simulink library "Contact_Forces_Lib"  (R2025a)
settings: Solver=ode45  StartTime=0.0  StopTime=10.0  RelTol=1e-3  EnableMultiTasking=on
undefined symbols (not defined in the file or in its folder): b_contact, custom_param_1, custom_param_2, Extr_Data_Ring, k_contact, l_cone, length_cylinder, length_tube, mu_kinetic, mu_static, pen_exponent, pen_full_damp_F, rad_s_cone, radius_cylinder, radius_tube, v_thr, X, Y, Z
libraries: nesl_utility x197, sm_lib x115, $bdroot x72, simulink x20, fl_lib x4
(part 1 of 12)
Description:
  | Simscape Multibody Contact Forces Library v5.0
  | Copyright 2014-2025 The MathWorks, Inc.
settings Model: Creator=smiller  LastModifiedBy=smiller
settings SolverCC: AlgebraicLoopSolver=TrustRegion
settings DataIOCC: LimitDataPoints=on  SaveFormat=Array  ReturnWorkspaceOutputs=off
settings OptimizationCC: ReuseModelBlockBuffer=off  LifeSpan=inf
settings DebuggingCC: SolverPrmCheckMsg=warning  UnconnectedInputMsg=warning  UnconnectedOutputMsg=warning  UnconnectedLineMsg=warning  AllowSymbolicDim=off  PregeneratedLibrarySubsystemCodeDiagnostic=none  SFUnexpectedBacktrackingDiag=warning  SFNoUnconditionalDefaultTransitionDiag=warning  SFExecutionAtInitializationDiag=none  ArithmeticOperatorsInVariantConditions=warning
settings HardwareCC: ProdBitPerPointer=32.0  ProdBitPerSizeT=32.0  ProdBitPerPtrDiffT=32.0  ProdLargestAtomicFloat=None  ProdIntDivRoundTo=Undefined  ProdEndianess=Unspecified  ProdWordSize=32.0  ProdHWDeviceType=32-bit Generic
settings ModelReferenceCC: EnableRefExpFcnMdlSchedulingChecks=on  PropagateSignalLabelsOutOfModel=off
settings SFSimCC: SimUseLocalCustomCode=off  CustomCodeUndefinedFunction=UseInterfaceOnly
settings RTWCC: RTWUseLocalCustomCode=off  GPUComputeCapability=3.5  DLArmComputeVersion=19.05
settings CodeAppCC: StateflowObjectComments=on
settings GRTTargetCC: TargetLangStandard=C89/C90 (ANSI)
settings ConfigComp: CovMetricSettings=dw  CovSaveCumulativeToWorkspaceVar=on  CovSaveSingleToWorkspaceVar=on  CovExternalEMLEnable=off  CovSFcnEnable=off

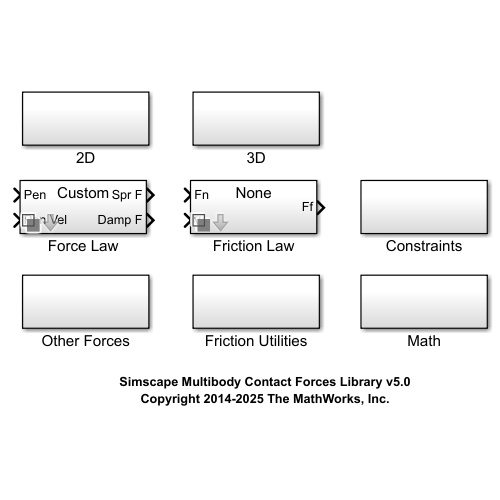
[thumbnail: Simulink's stored preview of the top-level diagram]
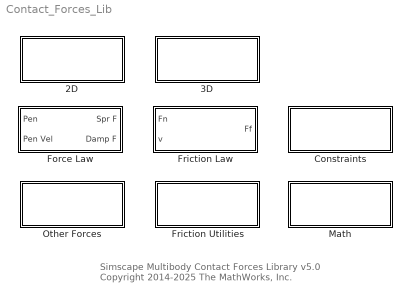
== system Contact_Forces_Lib ==
  note: Simscape Multibody Contact Forces Library v5.0
      | Copyright 2014-2025 The MathWorks, Inc.
  2D : Subsystem
  3D : Subsystem
  Constraints : Subsystem
  Force Law : Subsystem  Variant=on  VariantControlMode=label  LabelModeActiveChoice=Custom
  Friction Law : Subsystem  Variant=on  VariantControlMode=label  LabelModeActiveChoice=None
  Friction Utilities : Subsystem
  Math : Subsystem
  Other Forces : Subsystem

== system Contact_Forces_Lib/2D ==
  Circle to Circle Force : Subsystem  mask(Circle to Circle Force){cirB_rad=0.1, cirF_rad=0.1, active_angle=[-180 180], force_law=Linear, k_contact=1e4, b_contact=1e2, pen_full_damp_F=1e-4, pen_exponent=1, custom_param_1=1, custom_param_2=1, friction_law=None, mu_kinetic=0.5, mu_static=0.7, v_thr=0.001, vis_on=off, vis_opc_en=0, vis_len_cirBz=0.1, vis_len_cirBx=0.005, vis_len_cirFz=0.1, vis_len_cirFx=0.005, vis_clr=[0.9 0.2 0.2], vis_opc=0.7}
      mask prompts: cirB_rad "Base Radius (m)"; cirF_rad "Follower Radius (m)"; active_angle "Active Range (min, max angle (deg))"; force_law "Force Law"; k_contact "Contact Stiffness (N/m)"; b_contact "Contact Damping (N/(m/s))"; pen_full_damp_F "Penetration for full damping (m)"; pen_exponent "Penetration exponent (>=1)"; custom_param_1 "Custom Parameter 1"; custom_param_2 "Custom Parameter 2"; friction_law "Friction Law"; mu_kinetic "Coefficient of Kinetic Friction"; mu_static "Coefficient of Static Friction"; v_thr "Velocity Threshold (m/s)"; vis_on "Visualize Contact Surfaces"; vis_opc_en "Visualize Opacity Enable"; vis_clr "Color of Surface Element (RGB)"; vis_opc "Opacity of Surface Element (0-1)"
      mask help:
      | This subsystem implements a 2D contact force between two circles. It acts to repel frames CirB and CirF.
      |
      | Frames connected to ports:
      | 1. Located at center of circle
      | 2. Circle is in XY plane of frame
      | 3. Active range: counter-clockwise from -x axis of CirB
      |
      | Output signal is a bus with intermediate calculations and total force. Click Help for a diagram describing this force.
      mask init:
      | if strcmp(get_param(gcb,'force_law'),'Linear')
      |     set_param([gcb '/Force Law'],'OverrideUsingVariant','Linear');
      | elseif strcmp(get_param(gcb,'force_law'),'Nonlinear')
      |     set_param([gcb '/Force Law'],'OverrideUsingVariant','Nonlinear');
      | elseif strcmp(get_param(gcb,'force_law'),'Custom')
      |     set_param([gcb '/Force Law'],'OverrideUsingVariant','Custom');
      | end
      | 
      | if strcmp(get_param(gcb,'friction_law'),'None')
      |     set_param([gcb '/Ff/Friction Law'],'OverrideUsingVariant','None');
      | elseif strcmp(get_param(gcb,'friction_law'),'Stick-Slip Continuous')
      |     set_param([gcb '/Ff/Friction Law'],'OverrideUsingVariant','Stick_Slip_C');
      | end
      | 
      | if strcmp(get_param(gcb,'vis_on'),'on')
      |     vis_opc_en = 1;
      | elseif strcmp(get_param(gcb,'vis_on'),'off')
      |     vis_opc_en = 0;
      | end
      mask Help: web(which('Circle_to_Circle_Contact.html'));
      mask TypeOptions force_law: Linear | Nonlinear | Custom
      mask Callback force_law:
      | maskObj = Simulink.Mask.get(gcb);
      | pfd_h = maskObj.getParameter('pen_full_damp_F');
      | pex_h = maskObj.getParameter('pen_exponent');
      | cc1_h = maskObj.getParameter('custom_param_1');
      | cc2_h = maskObj.getParameter('custom_param_2');
      | if strcmp(get_param(gcb,'force_law'),'Linear')
      |     pfd_h.Visible = 'off';
      |     pex_h.Visible = 'off';
      |     cc1_h.Visible = 'off';
      |     cc2_h.Visible = 'off';
      | elseif strcmp(get_param(gcb,'force_law'),'Nonlinear')
      |     pfd_h.Visible = 'on';
      |     pex_h.Visible = 'on';
      |     cc1_h.Visible = 'off';
      |     cc2_h.Visible = 'off';
      | elseif strcmp(get_param(gcb,'force_law'),'Custom')
      |     pfd_h.Visible = 'off';
      |     pex_h.Visible = 'off';
      |     cc1_h.Visible = 'on';
      |     cc2_h.Visible = 'on';
      | end
      | 
      | clear maskObj pfd_h pex_h cc1_h cc2_h
      mask TypeOptions friction_law: None | Stick-Slip Continuous
      mask Callback friction_law:
      | maskObj = Simulink.Mask.get(gcb);
      | muk_h = maskObj.getParameter('mu_kinetic');
      | mus_h = maskObj.getParameter('mu_static');
      | vth_h = maskObj.getParameter('v_thr');
      | if strcmp(get_param(gcb,'friction_law'),'None')
      |     muk_h.Visible = 'off';
      |     mus_h.Visible = 'off';
      |     vth_h.Visible = 'off';
      | elseif strcmp(get_param(gcb,'friction_law'),'Stick-Slip Continuous')
      |     muk_h.Visible = 'on';
      |     mus_h.Visible = 'on';
      |     vth_h.Visible = 'on';
      | end
      | clear maskObj muk_h mus_h vth_h
      mask Callback vis_on:
      | maskObj = Simulink.Mask.get(gcb);
      | 
      | vis_len_prompt_h = maskObj.getDialogControl('vis_len_prompt');
      | vis_len_promptZaxis_h = maskObj.getDialogControl('vis_len_promptZaxis');
      | vis_len_promptXaxis_h = maskObj.getDialogControl('vis_len_promptXaxis');
      | vis_len_promptBase_h = maskObj.getDialogControl('vis_len_promptBase');
      | vis_len_promptFollower_h = maskObj.getDialogControl('vis_len_promptFollower');
      | vis_len_cirBz_h = maskObj.getParameter('vis_len_cirBz');
      | vis_len_cirBx_h = maskObj.getParameter('vis_len_cirBx');
      | vis_len_cirFz_h = maskObj.getParameter('vis_len_cirFz');
      | vis_len_cirFx_h = maskObj.getParameter('vis_len_cirFx');
      | vis_clr_h = maskObj.getParameter('vis_clr');
      | vis_opc_h = maskObj.getParameter('vis_opc');
      | 
      | temp_visCBstate = get_param(gcb,'vis_on');
      | vis_len_prompt_h.Visible = temp_visCBstate;
      | vis_len_promptZaxis_h.Visible = temp_visCBstate;
      | vis_len_promptXaxis_h.Visible = temp_visCBstate;
      | vis_len_promptBase_h.Visible = temp_visCBstate;
      | vis_len_promptFollower_h.Visible = temp_visCBstate;
      | vis_len_cirBz_h.Visible = temp_visCBstate;
      | vis_len_cirBx_h.Visible = temp_visCBstate;
      | vis_len_cirFz_h.Visible = temp_visCBstate;
      | vis_len_cirFx_h.Visible = temp_visCBstate;
      | vis_clr_h.Visible = temp_visCBstate;
      | vis_opc_h.Visible = temp_visCBstate;
      | 
      | clear maskObj vis_clr_h vis_opc_h
      | clear vis_len_prompt_h temp_visCBstate
      | clear vis_len_promptZaxis_h vis_len_promptXaxis_h
      | clear vis_len_promptBase_h vis_len_promptFollower_h
      | clear vis_len_cirBz_h vis_len_cirBx_h
      | clear vis_len_cirFz_h vis_len_cirFx_h
      mask DialogControl Dim_Cont Prompt: Dimensions
      mask DialogControl Con_cont Prompt: Contact
      mask DialogControl Fri_Cont Prompt: Friction
      mask DialogControl Container11 Prompt: Visual
      mask DialogControl vis_len_prompt Prompt: Length of Surface
      mask DialogControl vis_len_promptZaxis Prompt: Z-Axis (m)
      mask DialogControl vis_len_promptXaxis Prompt: X-Axis (m)
      mask DialogControl vis_len_promptBase Prompt: Base
      mask DialogControl vis_len_promptFollower Prompt: Follower
      mask Display: image('Circle_to_Circle_Contact_IMAGE.jpg');
  Circle to Circle Force Enabled : Subsystem  mask(Circle to Circle Force Enabled){cirB_rad=0.1, cirF_rad=0.1, active_angle=[-180 180], force_law=Linear, k_contact=1e4, b_contact=1e2, pen_full_damp_F=1e-4, pen_exponent=1, custom_param_1=1, custom_param_2=1, friction_law=None, mu_kinetic=0.5, mu_static=0.7, v_thr=0.001, vis_on=off, vis_opc_en=0, vis_len_cirBz=0.1, vis_len_cirBx=0.005, vis_len_cirFz=0.1, vis_len_cirFx=0.005, vis_clr=[0.9 0.2 0.2], vis_opc=0.7}
      mask prompts: cirB_rad "Base Radius (m)"; cirF_rad "Follower Radius (m)"; active_angle "Active Range (min, max angle (deg))"; force_law "Force Law"; k_contact "Contact Stiffness (N/m)"; b_contact "Contact Damping (N/(m/s))"; pen_full_damp_F "Penetration for full damping (m)"; pen_exponent "Penetration exponent (>=1)"; custom_param_1 "Custom Parameter 1"; custom_param_2 "Custom Parameter 2"; friction_law "Friction Law"; mu_kinetic "Coefficient of Kinetic Friction"; mu_static "Coefficient of Static Friction"; v_thr "Velocity Threshold (m/s)"; vis_on "Visualize Contact Surfaces"; vis_opc_en "Visualize Opacity Enable"; vis_clr "Color of Surface Element (RGB)"; vis_opc "Opacity of Surface Element (0-1)"
      mask help:
      | This subsystem implements a 2D contact force between two circles. It acts to repel frames CirB and CirF.
      |
      | Frames connected to ports:
      | 1. Located at center of circle
      | 2. Circle is in XY plane of frame
      | 3. Active range: counter-clockwise from -x axis of CirB
      |
      | Input signal is a bus with signals that control aspects of the force, including enable/disable. Output signal is a bus with intermediate calculations and total force. Click Help for a diagram describing this force.
      mask init: same as Contact_Forces_Lib/2D/Circle to Circle Force
      mask Help: web(which('Circle_to_Circle_Contact.html'));
      mask TypeOptions force_law: Linear | Nonlinear | Custom
      mask Callback force_law:
      | maskObj = Simulink.Mask.get(gcb);
      | pfd_h = maskObj.getParameter('pen_full_damp_F');
      | pex_h = maskObj.getParameter('pen_exponent');
      | cc1_h = maskObj.getParameter('custom_param_1');
      | cc2_h = maskObj.getParameter('custom_param_2');
      | if strcmp(get_param(gcb,'force_law'),'Linear')
      |     pfd_h.Visible = 'off';
      |     pex_h.Visible = 'off';
      |     cc1_h.Visible = 'off';
      |     cc2_h.Visible = 'off';
      | elseif strcmp(get_param(gcb,'force_law'),'Nonlinear')
      |     pfd_h.Visible = 'on';
      |     pex_h.Visible = 'on';
      |     cc1_h.Visible = 'off';
      |     cc2_h.Visible = 'off';
      | elseif strcmp(get_param(gcb,'force_law'),'Custom')
      |     pfd_h.Visible = 'off';
      |     pex_h.Visible = 'off';
      |     cc1_h.Visible = 'on';
      |     cc2_h.Visible = 'on';
      | end
      | 
      | clear maskObj pfd_h pex_h cc1_h cc2_h
      mask TypeOptions friction_law: None | Stick-Slip Continuous
      mask Callback friction_law:
      | maskObj = Simulink.Mask.get(gcb);
      | muk_h = maskObj.getParameter('mu_kinetic');
      | mus_h = maskObj.getParameter('mu_static');
      | vth_h = maskObj.getParameter('v_thr');
      | if strcmp(get_param(gcb,'friction_law'),'None')
      |     muk_h.Visible = 'off';
      |     mus_h.Visible = 'off';
      |     vth_h.Visible = 'off';
      | elseif strcmp(get_param(gcb,'friction_law'),'Stick-Slip Continuous')
      |     muk_h.Visible = 'on';
      |     mus_h.Visible = 'on';
      |     vth_h.Visible = 'on';
      | end
      | clear maskObj muk_h mus_h vth_h
      mask Callback vis_on:
      | maskObj = Simulink.Mask.get(gcb);
      | 
      | vis_len_prompt_h = maskObj.getDialogControl('vis_len_prompt');
      | vis_len_promptZaxis_h = maskObj.getDialogControl('vis_len_promptZaxis');
      | vis_len_promptXaxis_h = maskObj.getDialogControl('vis_len_promptXaxis');
      | vis_len_promptBase_h = maskObj.getDialogControl('vis_len_promptBase');
      | vis_len_promptFollower_h = maskObj.getDialogControl('vis_len_promptFollower');
      | vis_len_cirBz_h = maskObj.getParameter('vis_len_cirBz');
      | vis_len_cirBx_h = maskObj.getParameter('vis_len_cirBx');
      | vis_len_cirFz_h = maskObj.getParameter('vis_len_cirFz');
      | vis_len_cirFx_h = maskObj.getParameter('vis_len_cirFx');
      | vis_clr_h = maskObj.getParameter('vis_clr');
      | vis_opc_h = maskObj.getParameter('vis_opc');
      | 
      | temp_visCBstate = get_param(gcb,'vis_on');
      | vis_len_prompt_h.Visible = temp_visCBstate;
      | vis_len_promptZaxis_h.Visible = temp_visCBstate;
      | vis_len_promptXaxis_h.Visible = temp_visCBstate;
      | vis_len_promptBase_h.Visible = temp_visCBstate;
      | vis_len_promptFollower_h.Visible = temp_visCBstate;
      | vis_len_cirBz_h.Visible = temp_visCBstate;
      | vis_len_cirBx_h.Visible = temp_visCBstate;
      | vis_len_cirFz_h.Visible = temp_visCBstate;
      | vis_len_cirFx_h.Visible = temp_visCBstate;
      | vis_clr_h.Visible = temp_visCBstate;
      | vis_opc_h.Visible = temp_visCBstate;
      | 
      | clear maskObj vis_clr_h vis_opc_h
      | clear vis_len_prompt_h temp_visCBstate
      | clear vis_len_promptZaxis_h vis_len_promptXaxis_h
      | clear vis_len_promptBase_h vis_len_promptFollower_h
      | clear vis_len_cirBz_h vis_len_cirBx_h
      | clear vis_len_cirFz_h vis_len_cirFx_h
      mask DialogControl Dim_Cont Prompt: Dimensions
      mask DialogControl Con_cont Prompt: Contact
      mask DialogControl Fri_Cont Prompt: Friction
      mask DialogControl Container11 Prompt: Visual
      mask DialogControl vis_len_prompt Prompt: Length of Surface
      mask DialogControl vis_len_promptZaxis Prompt: Z-Axis (m)
      mask DialogControl vis_len_promptXaxis Prompt: X-Axis (m)
      mask DialogControl vis_len_promptBase Prompt: Base
      mask DialogControl vis_len_promptFollower Prompt: Follower
      mask Display: image('Circle_to_Circle_Contact_Enabled_IMAGE.jpg');
  Circle to Finite Line Force : Subsystem  mask(Circle on Finite Line Force){circle_rad=0.2, line_depth=0.05/2, line_length=5, force_law=Linear, k_contact=1e5, b_contact=1e2, pen_full_damp_F=1e-4, pen_exponent=1, custom_param_1=1, custom_param_2=1, friction_law=None, mu_kinetic=0.5, mu_static=0.7, v_thr=0.001, vis_on=off, vis_opc_en=0, vis_len_linBz=0.1, vis_len_linBx=0.005, vis_len_cirFz=0.1, vis_len_cirFx=0.005, vis_clr=[0.9 0.2 0.2], vis_opc=0.7}
      mask prompts: circle_rad "Circle Radius (m)"; line_depth "Line Depth to Reference Frame (m)"; line_length "Line Length (m)"; force_law "Force Law"; k_contact "Contact Stiffness (N/m)"; b_contact "Contact Damping (N/(m/s))"; pen_full_damp_F "Penetration for full damping (m)"; pen_exponent "Penetration exponent (>=1)"; custom_param_1 "Custom Parameter 1"; custom_param_2 "Custom Parameter 2"; friction_law "Friction Law"; mu_kinetic "Coefficient of Kinetic Friction"; mu_static "Coefficient of Static Friction"; v_thr "Velocity Threshold (m/s)"; vis_on "Visualize Contact Surface"; vis_opc_en "Visualize Opacity Enable"; vis_clr "Color of Surface Element (RGB)"; vis_opc "Opacity of Surface Element (0-1)"
      mask help:
      | This subsystem implements a 2D contact force between a circle and a finite line.  The force is active above and below the line.
      |
      | Frame connected to LinB port:
      | 1. Located at midpoint of line.
      | 2. X-axis is normal to the finite line.
      | 3. Y-axis is along the finite line.
      |
      | Frame connected to the CirF port:
      | 1. Z-axis aligned with frame attached to LinB port.
      |
      | Output signal is a bus with intermediate calculations and total force. Click Help for a diagram describing this force.
      mask init:
      | if strcmp(get_param(gcb,'force_law'),'Linear')
      |     set_param([gcb '/Forces/Force Law'],'OverrideUsingVariant','Linear');
      | elseif strcmp(get_param(gcb,'force_law'),'Nonlinear')
      |     set_param([gcb '/Forces/Force Law'],'OverrideUsingVariant','Nonlinear');
      | elseif strcmp(get_param(gcb,'force_law'),'Custom')
      |     set_param([gcb '/Forces/Force Law'],'OverrideUsingVariant','Custom');
      | end
      | 
      | if strcmp(get_param(gcb,'friction_law'),'None')
      |     set_param([gcb '/Forces/Resolve Forces/Friction/Friction Law'],'OverrideUsingVariant','None');
      | elseif strcmp(get_param(gcb,'friction_law'),'Stick-Slip Continuous')
      |     set_param([gcb '/Forces/Resolve Forces/Friction/Friction Law'],'OverrideUsingVariant','Stick_Slip_C');
      | end
      | 
      | if strcmp(get_param(gcb,'vis_on'),'on')
      |     vis_opc_en = 1;
      | elseif strcmp(get_param(gcb,'vis_on'),'off')
      |     vis_opc_en = 0;
      | end
      mask Help: web(which('Circle_to_Finite_Line_Contact.html'));
      mask TypeOptions force_law: Linear | Nonlinear | Custom
      mask Callback force_law:
      | %maskStr = get_param(gcb,'MaskValues');
      | maskObj = Simulink.Mask.get(gcb);
      | pfd_h = maskObj.getParameter('pen_full_damp_F');
      | pex_h = maskObj.getParameter('pen_exponent');
      | cc1_h = maskObj.getParameter('custom_param_1');
      | cc2_h = maskObj.getParameter('custom_param_2');
      | if strcmp(get_param(gcb,'force_law'),'Linear')
      |     pfd_h.Visible = 'off';
      |     pex_h.Visible = 'off';
      |     cc1_h.Visible = 'off';
      |     cc2_h.Visible = 'off';
      | %    set_param(gcb,'MaskVisibilities',{'on' 'on' 'on' 'on' 'on' 'off' 'off' 'off' 'off'});
      | %    set_param(gcb,'MaskVisibilities',{'on' 'on' 'on' 'on' 'on' 'off' 'off' 'off' 'off'});
      | elseif strcmp(get_param(gcb,'force_law'),'Nonlinear')
      |     pfd_h.Visible = 'on';
      |     pex_h.Visible = 'on';
      |     cc1_h.Visible = 'off';
      |     cc2_h.Visible = 'off';
      |     %set_param(gcb,'MaskVisibilities',{'on' 'on' 'on' 'on' 'on' 'on' 'on' 'off' 'off'});
      | elseif strcmp(get_param(gcb,'force_law'),'Custom')
      |     pfd_h.Visible = 'off';
      |     pex_h.Visible = 'off';
      |     cc1_h.Visible = 'on';
      |     cc2_h.Visible = 'on';
      |     %set_param(gcb,'MaskVisibilities',{'on' 'on' 'on' 'on' 'on' 'off' 'off' 'on' 'on'});
      | end
      | %clear maskObj
      | 
      | %maskObj = Simulink.Mask.get(gcb);
      | %if strcmp(get_param(gcb,'x'),'on')
      | %else
      | %    yh.Visible = 'off';
      | %end
      mask TypeOptions friction_law: None | Stick-Slip Continuous
      mask Callback friction_law:
      | maskObj = Simulink.Mask.get(gcb);
      | muk_h = maskObj.getParameter('mu_kinetic');
      | mus_h = maskObj.getParameter('mu_static');
      | vth_h = maskObj.getParameter('v_thr');
      | if strcmp(get_param(gcb,'friction_law'),'None')
      |     muk_h.Visible = 'off';
      |     mus_h.Visible = 'off';
      |     vth_h.Visible = 'off';
      | elseif strcmp(get_param(gcb,'friction_law'),'Stick-Slip Continuous')
      |     muk_h.Visible = 'on';
      |     mus_h.Visible = 'on';
      |     vth_h.Visible = 'on';
      | end
      | clear maskObj
      mask Callback vis_on:
      | maskObj = Simulink.Mask.get(gcb);
      | vis_len_prompt_h = maskObj.getDialogControl('vis_len_prompt');
      | vis_len_promptZaxis_h = maskObj.getDialogControl('vis_len_promptZaxis');
      | vis_len_promptXaxis_h = maskObj.getDialogControl('vis_len_promptXaxis');
      | vis_len_promptBase_h = maskObj.getDialogControl('vis_len_promptBase');
      | vis_len_promptFollower_h = maskObj.getDialogControl('vis_len_promptFollower');
      | vis_len_linBz_h = maskObj.getParameter('vis_len_linBz');
      | vis_len_linBx_h = maskObj.getParameter('vis_len_linBx');
      | vis_len_cirFz_h = maskObj.getParameter('vis_len_cirFz');
      | vis_len_cirFx_h = maskObj.getParameter('vis_len_cirFx');
      | vis_clr_h = maskObj.getParameter('vis_clr');
      | vis_opc_h = maskObj.getParameter('vis_opc');
      | 
      | temp_visCBstate = get_param(gcb,'vis_on');
      | vis_len_prompt_h.Visible = temp_visCBstate;
      | vis_len_promptZaxis_h.Visible = temp_visCBstate;
      | vis_len_promptXaxis_h.Visible = temp_visCBstate;
      | vis_len_promptBase_h.Visible = temp_visCBstate;
      | vis_len_promptFollower_h.Visible = temp_visCBstate;
      | vis_len_linBz_h.Visible = temp_visCBstate;
      | vis_len_linBx_h.Visible = temp_visCBstate;
      | vis_len_cirFz_h.Visible = temp_visCBstate;
      | vis_len_cirFx_h.Visible = temp_visCBstate;
      | vis_clr_h.Visible = temp_visCBstate;
      | vis_opc_h.Visible = temp_visCBstate;
      | 
      | clear maskObj vis_len_h vis_clr_h vis_opc_h
      | clear temp_visCBstate
      | clear vis_len_prompt_h vis_len_promptZaxis_h vis_len_promptXaxis_h
      | clear vis_len_promptBase_h vis_len_promptFollower_h
      | clear vis_len_linBz_h vis_len_linBx_h
      | clear vis_len_cirFz_h vis_len_cirFx_h
      mask DialogControl Dim_Cont Prompt: Dimensions
      mask DialogControl Con_Cont Prompt: Contact
      mask DialogControl Fri_Cont Prompt: Friction
      mask DialogControl Container9 Prompt: Visual
      mask DialogControl vis_len_prompt Prompt: Length of Surface
      mask DialogControl vis_len_promptZaxis Prompt: Z-Axis (m)
      mask DialogControl vis_len_promptXaxis Prompt: X-Axis (m)
      mask DialogControl vis_len_promptBase Prompt: Base (Line)
      mask DialogControl vis_len_promptFollower Prompt: Follower (Cir)
      mask Display: image('Circle_to_Finite_Line_Contact_IMAGE.jpg');
  Circle to Finite Line Force Enabled : Subsystem  mask(Circle on Finite Line Force Enabled){circle_rad=0.2, line_depth=0.05/2, line_length=5, force_law=Linear, k_contact=1e5, b_contact=1e2, pen_full_damp_F=1e-4, pen_exponent=1, custom_param_1=1, custom_param_2=1, friction_law=None, mu_kinetic=0.5, mu_static=0.7, v_thr=0.001, vis_on=off, vis_opc_en=0, vis_len_linBz=0.1, vis_len_linBx=0.005, vis_len_cirFz=0.1, vis_len_cirFx=0.005, vis_clr=[0.9 0.2 0.2], vis_opc=0.7}
      mask prompts: circle_rad "Circle Radius (m)"; line_depth "Line Depth to Reference Frame (m)"; line_length "Line Length (m)"; force_law "Force Law"; k_contact "Contact Stiffness (N/m)"; b_contact "Contact Damping (N/(m/s))"; pen_full_damp_F "Penetration for full damping (m)"; pen_exponent "Penetration exponent (>=1)"; custom_param_1 "Custom Parameter 1"; custom_param_2 "Custom Parameter 2"; friction_law "Friction Law"; mu_kinetic "Coefficient of Kinetic Friction"; mu_static "Coefficient of Static Friction"; v_thr "Velocity Threshold (m/s)"; vis_on "Visualize Contact Surface"; vis_opc_en "Visualize Opacity Enable"; vis_clr "Color of Surface Element (RGB)"; vis_opc "Opacity of Surface Element (0-1)"
      mask help:
      | This subsystem implements a 2D contact force between a circle and a finite line.  The force is active above and below the line.
      |
      | Frame connected to LinB port:
      | 1. Located at midpoint of line.
      | 2. X-axis is normal to the finite line.
      | 3. Y-axis is along the finite line.
      |
      | Frame connected to the CirF port:
      | 1. Z-axis aligned with frame attached to LinB port.
      |
      | Input signal is a bus with signals that control aspects of the force, including enable/disable. Output signal is a bus with intermediate calculations and total force. Click Help for a diagram describing this force.
      mask init: same as Contact_Forces_Lib/2D/Circle to Finite Line Force
      mask Help: web(which('Circle_to_Finite_Line_Contact.html'));
      mask TypeOptions force_law: Linear | Nonlinear | Custom
      mask Callback force_law:
      | %maskStr = get_param(gcb,'MaskValues');
      | maskObj = Simulink.Mask.get(gcb);
      | pfd_h = maskObj.getParameter('pen_full_damp_F');
      | pex_h = maskObj.getParameter('pen_exponent');
      | cc1_h = maskObj.getParameter('custom_param_1');
      | cc2_h = maskObj.getParameter('custom_param_2');
      | if strcmp(get_param(gcb,'force_law'),'Linear')
      |     pfd_h.Visible = 'off';
      |     pex_h.Visible = 'off';
      |     cc1_h.Visible = 'off';
      |     cc2_h.Visible = 'off';
      | %    set_param(gcb,'MaskVisibilities',{'on' 'on' 'on' 'on' 'on' 'off' 'off' 'off' 'off'});
      | %    set_param(gcb,'MaskVisibilities',{'on' 'on' 'on' 'on' 'on' 'off' 'off' 'off' 'off'});
      | elseif strcmp(get_param(gcb,'force_law'),'Nonlinear')
      |     pfd_h.Visible = 'on';
      |     pex_h.Visible = 'on';
      |     cc1_h.Visible = 'off';
      |     cc2_h.Visible = 'off';
      |     %set_param(gcb,'MaskVisibilities',{'on' 'on' 'on' 'on' 'on' 'on' 'on' 'off' 'off'});
      | elseif strcmp(get_param(gcb,'force_law'),'Custom')
      |     pfd_h.Visible = 'off';
      |     pex_h.Visible = 'off';
      |     cc1_h.Visible = 'on';
      |     cc2_h.Visible = 'on';
      |     %set_param(gcb,'MaskVisibilities',{'on' 'on' 'on' 'on' 'on' 'off' 'off' 'on' 'on'});
      | end
      | %clear maskObj
      | 
      | %maskObj = Simulink.Mask.get(gcb);
      | %if strcmp(get_param(gcb,'x'),'on')
      | %else
      | %    yh.Visible = 'off';
      | %end
      mask TypeOptions friction_law: None | Stick-Slip Continuous
      mask Callback friction_law:
      | maskObj = Simulink.Mask.get(gcb);
      | muk_h = maskObj.getParameter('mu_kinetic');
      | mus_h = maskObj.getParameter('mu_static');
      | vth_h = maskObj.getParameter('v_thr');
      | if strcmp(get_param(gcb,'friction_law'),'None')
      |     muk_h.Visible = 'off';
      |     mus_h.Visible = 'off';
      |     vth_h.Visible = 'off';
      | elseif strcmp(get_param(gcb,'friction_law'),'Stick-Slip Continuous')
      |     muk_h.Visible = 'on';
      |     mus_h.Visible = 'on';
      |     vth_h.Visible = 'on';
      | end
      | clear maskObj
      mask Callback vis_on:
      | maskObj = Simulink.Mask.get(gcb);
      | vis_len_prompt_h = maskObj.getDialogControl('vis_len_prompt');
      | vis_len_promptZaxis_h = maskObj.getDialogControl('vis_len_promptZaxis');
      | vis_len_promptXaxis_h = maskObj.getDialogControl('vis_len_promptXaxis');
      | vis_len_promptBase_h = maskObj.getDialogControl('vis_len_promptBase');
      | vis_len_promptFollower_h = maskObj.getDialogControl('vis_len_promptFollower');
      | vis_len_linBz_h = maskObj.getParameter('vis_len_linBz');
      | vis_len_linBx_h = maskObj.getParameter('vis_len_linBx');
      | vis_len_cirFz_h = maskObj.getParameter('vis_len_cirFz');
      | vis_len_cirFx_h = maskObj.getParameter('vis_len_cirFx');
      | vis_clr_h = maskObj.getParameter('vis_clr');
      | vis_opc_h = maskObj.getParameter('vis_opc');
      | 
      | temp_visCBstate = get_param(gcb,'vis_on');
      | vis_len_prompt_h.Visible = temp_visCBstate;
      | vis_len_promptZaxis_h.Visible = temp_visCBstate;
      | vis_len_promptXaxis_h.Visible = temp_visCBstate;
      | vis_len_promptBase_h.Visible = temp_visCBstate;
      | vis_len_promptFollower_h.Visible = temp_visCBstate;
      | vis_len_linBz_h.Visible = temp_visCBstate;
      | vis_len_linBx_h.Visible = temp_visCBstate;
      | vis_len_cirFz_h.Visible = temp_visCBstate;
      | vis_len_cirFx_h.Visible = temp_visCBstate;
      | vis_clr_h.Visible = temp_visCBstate;
      | vis_opc_h.Visible = temp_visCBstate;
      | 
      | clear maskObj vis_len_h vis_clr_h vis_opc_h
      | clear temp_visCBstate
      | clear vis_len_prompt_h vis_len_promptZaxis_h vis_len_promptXaxis_h
      | clear vis_len_promptBase_h vis_len_promptFollower_h
      | clear vis_len_linBz_h vis_len_linBx_h
      | clear vis_len_cirFz_h vis_len_cirFx_h
      mask DialogControl Dim_Cont Prompt: Dimensions
      mask DialogControl Con_Cont Prompt: Contact
      mask DialogControl Fri_Cont Prompt: Friction
      mask DialogControl Container9 Prompt: Visual
      mask DialogControl vis_len_prompt Prompt: Length of Surface
      mask DialogControl vis_len_promptZaxis Prompt: Z-Axis (m)
      mask DialogControl vis_len_promptXaxis Prompt: X-Axis (m)
      mask DialogControl vis_len_promptBase Prompt: Base (Line)
      mask DialogControl vis_len_promptFollower Prompt: Follower (Cir)
      mask Display: image('Circle_to_Finite_Line_Contact_Enabled_IMAGE.jpg');
  Circle to Hole Force : Subsystem  mask(Circle to Hole Force){k_contact=-1e4, b_contact=10, max_frame_sep=0.1079, active_angle=[-180 180], h_deadzone=0.6667}
      mask prompts: k_contact "Attraction Stiffness (N/m)"; b_contact "Attraction Damping (N/(m/s))"; max_frame_sep "Maximum Frame Separation (m)"; active_angle "Active Range (min, max angle relative to frame CirB (deg))"; h_deadzone "Hole Deadzone (% of radius)"
      mask help: This subsystem implements an attraction force between a circle and a hole. This force operates on the XY plane of the CirB frame. A deadzone is applied to the stiffness force at the center of the hole to allow the circle to come to rest.
      mask Display: image('Circle_to_Hole_Attraction_IMAGE.jpg');
  Circle to Ring Force : Subsystem  mask(Circle to Ring Force){radius_circle=0.05, radius_ring=0.07, d_ring=0.02, active_angle=[-120 120], force_law=Linear, k_contact=1e4, b_contact=1e2, pen_full_damp_F=1e-4, pen_exponent=1, custom_param_1=1, custom_param_2=1, friction_law=Stick-Slip Continuous, mu_kinetic=0.1, mu_static=0.2, v_thr=0.001, vis_on=off, vis_opc_en=0, vis_len_rinBz=0.05*1.05, vis_len_rinBx=0.08*0.05, vis_len_cirFz=0.05*1.05, vis_len_cirFx=0.05*0.05, vis_clr=[0.9 0.2 0.2], vis_opc=0.7}
      mask prompts: radius_circle "Circle Radius (CirF) (m)"; radius_ring "Ring Radius (RinB) (m)"; d_ring "Ring Thickness (RinB) (m)"; active_angle "Active Range (min, max angle (deg))"; force_law "Force Law"; k_contact "Contact Stiffness (N/m)"; b_contact "Contact Damping (N/(m/s))"; pen_full_damp_F "Penetration for full damping (m)"; pen_exponent "Penetration exponent (>=1)"; custom_param_1 "Custom Parameter 1"; custom_param_2 "Custom Parameter 2"; friction_law "Friction Law"; mu_kinetic "Coefficient of Kinetic Friction"; mu_static "Coefficient of Static Friction"; v_thr "Velocity Threshold (m/s)"; vis_on "Visualize Contact Surface"; vis_opc_en "Visualize Opacity Enable"; vis_clr "Color of Visual Element (RGB)"; vis_opc "Opacity of Visual Element (0-1)"
      mask help:
      | This subsystem implements a 2D contact force between a circle and a ring.
      | The force is active on the outside and the inside of the ring.
      |
      | Frames connected to ports:
      | 1. Located at center of circle/ring
      | 2. Circle/Ring is in XY plane of frame
      | 3. Active range: relative to +x axis of RinB [-180 180]
      |
      | Output signal is a bus with intermediate calculations and total force. Click Help for a diagram describing this force.
      mask init:
      | if strcmp(get_param(gcb,'force_law'),'Linear')
      |     set_param([gcb '/Forces/Force Law'],'OverrideUsingVariant','Linear');
      | elseif strcmp(get_param(gcb,'force_law'),'Nonlinear')
      |     set_param([gcb '/Forces/Force Law'],'OverrideUsingVariant','Nonlinear');
      | elseif strcmp(get_param(gcb,'force_law'),'Custom')
      |     set_param([gcb '/Forces/Force Law'],'OverrideUsingVariant','Custom');
      | end
      | 
      | if strcmp(get_param(gcb,'friction_law'),'None')
      |     set_param([gcb '/Forces/Ff/Friction Law'],'OverrideUsingVariant','None');
      | elseif strcmp(get_param(gcb,'friction_law'),'Stick-Slip Continuous')
      |     set_param([gcb '/Forces/Ff/Friction Law'],'OverrideUsingVariant','Stick_Slip_C');
      | end
      | 
      | if strcmp(get_param(gcb,'vis_on'),'on')
      |     vis_opc_en = 1;
      | elseif strcmp(get_param(gcb,'vis_on'),'off')
      |     vis_opc_en = 0;
      | end
      mask Help: web(which('Circle_to_Ring_Contact.html'));
      mask TypeOptions force_law: Linear | Nonlinear | Custom
      mask Callback force_law:
      | %maskStr = get_param(gcb,'MaskValues');
      | maskObj = Simulink.Mask.get(gcb);
      | pfd_h = maskObj.getParameter('pen_full_damp_F');
      | pex_h = maskObj.getParameter('pen_exponent');
      | cc1_h = maskObj.getParameter('custom_param_1');
      | cc2_h = maskObj.getParameter('custom_param_2');
      | if strcmp(get_param(gcb,'force_law'),'Linear')
      |     pfd_h.Visible = 'off';
      |     pex_h.Visible = 'off';
      |     cc1_h.Visible = 'off';
      |     cc2_h.Visible = 'off';
      | %    set_param(gcb,'MaskVisibilities',{'on' 'on' 'on' 'on' 'on' 'off' 'off' 'off' 'off'});
      | %    set_param(gcb,'MaskVisibilities',{'on' 'on' 'on' 'on' 'on' 'off' 'off' 'off' 'off'});
      | elseif strcmp(get_param(gcb,'force_law'),'Nonlinear')
      |     pfd_h.Visible = 'on';
      |     pex_h.Visible = 'on';
      |     cc1_h.Visible = 'off';
      |     cc2_h.Visible = 'off';
      |     %set_param(gcb,'MaskVisibilities',{'on' 'on' 'on' 'on' 'on' 'on' 'on' 'off' 'off'});
      | elseif strcmp(get_param(gcb,'force_law'),'Custom')
      |     pfd_h.Visible = 'off';
      |     pex_h.Visible = 'off';
      |     cc1_h.Visible = 'on';
      |     cc2_h.Visible = 'on';
      |     %set_param(gcb,'MaskVisibilities',{'on' 'on' 'on' 'on' 'on' 'off' 'off' 'on' 'on'});
      | end
      | %clear maskObj
      | 
      | %maskObj = Simulink.Mask.get(gcb);
      | %if strcmp(get_param(gcb,'x'),'on')
      | %else
      | %    yh.Visible = 'off';
      | %end
      mask TypeOptions friction_law: None | Stick-Slip Continuous
      mask Callback friction_law:
      | maskObj = Simulink.Mask.get(gcb);
      | muk_h = maskObj.getParameter('mu_kinetic');
      | mus_h = maskObj.getParameter('mu_static');
      | vth_h = maskObj.getParameter('v_thr');
      | if strcmp(get_param(gcb,'friction_law'),'None')
      |     muk_h.Visible = 'off';
      |     mus_h.Visible = 'off';
      |     vth_h.Visible = 'off';
      | elseif strcmp(get_param(gcb,'friction_law'),'Stick-Slip Continuous')
      |     muk_h.Visible = 'on';
      |     mus_h.Visible = 'on';
      |     vth_h.Visible = 'on';
      | end
      | clear maskObj
      mask Callback vis_on:
      | maskObj = Simulink.Mask.get(gcb);
      | 
      | vis_len_prompt_h = maskObj.getDialogControl('vis_len_prompt');
      | vis_len_promptZaxis_h = maskObj.getDialogControl('vis_len_promptZaxis');
      | vis_len_promptXaxis_h = maskObj.getDialogControl('vis_len_promptXaxis');
      | vis_len_promptBase_h = maskObj.getDialogControl('vis_len_promptBase');
      | vis_len_promptFollower_h = maskObj.getDialogControl('vis_len_promptFollower');
      | vis_len_rinBz_h = maskObj.getParameter('vis_len_rinBz');
      | vis_len_rinBx_h = maskObj.getParameter('vis_len_rinBx');
      | vis_len_cirFz_h = maskObj.getParameter('vis_len_cirFz');
      | vis_len_cirFx_h = maskObj.getParameter('vis_len_cirFx');
      | vis_clr_h = maskObj.getParameter('vis_clr');
      | vis_opc_h = maskObj.getParameter('vis_opc');
      | 
      | temp_visCBstate = get_param(gcb,'vis_on');
      | vis_len_prompt_h.Visible = temp_visCBstate;
      | vis_len_promptZaxis_h.Visible = temp_visCBstate;
      | vis_len_promptXaxis_h.Visible = temp_visCBstate;
      | vis_len_promptBase_h.Visible = temp_visCBstate;
      | vis_len_promptFollower_h.Visible = temp_visCBstate;
      | vis_len_rinBz_h.Visible = temp_visCBstate;
      | vis_len_rinBx_h.Visible = temp_visCBstate;
      | vis_len_cirFz_h.Visible = temp_visCBstate;
      | vis_len_cirFx_h.Visible = temp_visCBstate;
      | vis_clr_h.Visible = temp_visCBstate;
      | vis_opc_h.Visible = temp_visCBstate;
      | 
      | clear maskObj vis_clr_h vis_opc_h
      | clear vis_len_prompt_h temp_visCBstate
      | clear vis_len_promptZaxis_h vis_len_promptXaxis_h
      | clear vis_len_promptBase_h vis_len_promptFollower_h
      | clear vis_len_rinBz_h vis_len_rinBx_h
      | clear vis_len_cirFz_h vis_len_cirFx_h
      mask DialogControl Dim_Cont Prompt: Dimensions
      mask DialogControl Con_cont Prompt: Contact
      mask DialogControl Fri_Cont Prompt: Friction
      mask DialogControl Container9 Prompt: Visual
      mask DialogControl vis_len_prompt Prompt: Length of Surface
      mask DialogControl vis_len_promptZaxis Prompt: Z-Axis (m)
      mask DialogControl vis_len_promptXaxis Prompt: X-Axis (m)
      mask DialogControl vis_len_promptBase Prompt: Base (Ring)
      mask DialogControl vis_len_promptFollower Prompt: Follower (Cir)
      mask Display: image('Circle_to_Ring_Contact_IMAGE.jpg');
  Composite Forces : Subsystem
